simulink model "baseline"  (R2025b)
settings: Solver=ode45  StartTime=0.0  StopTime=0.1  MaxStep=1e-5  RelTol=1e-8  AbsTol=1e-10
model workspace (MAT data in the model file):
  F = 0.008
  J = 0.003
  L = 0.0085
  Rs = 0.2
  Udc = 250
  p = 4
  psi = 0.175
Description:
  | Lumped AFPM equivalent with ideal complementary gates [A+ A- B+ B- C+ C-]. w_ref is a test interface only.
settings Model: Creator=A  LastModifiedBy=A

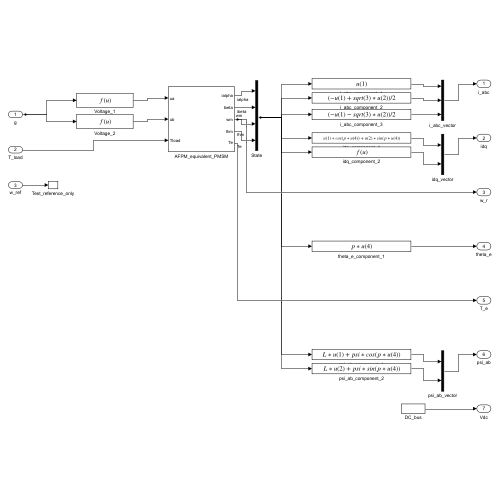
[thumbnail: Simulink's stored preview of the top-level diagram]
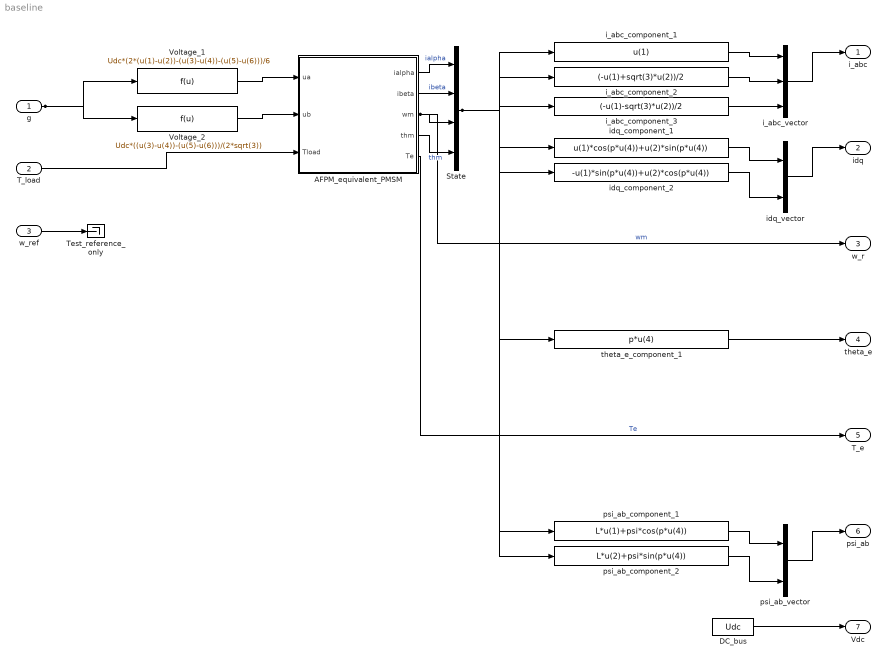
== system baseline ==
  g : Inport  Unit=1  PortDimensions=6
  T_load : Inport  Port=2  Unit=N*m  PortDimensions=1
  w_ref : Inport  Port=3  Unit=rpm  PortDimensions=1
  AFPM_equivalent_PMSM : Subsystem
  DC_bus : Constant  Value=Udc
  State : Mux
  Test_reference_only : Terminator
  Voltage_1 : Fcn  Expr=Udc*(2*(u(1)-u(2))-(u(3)-u(4))-(u(5)-u(6)))/6
  Voltage_2 : Fcn  Expr=Udc*((u(3)-u(4))-(u(5)-u(6)))/(2*sqrt(3))
  i_abc_component_1 : Fcn  Expr=u(1)
  i_abc_component_2 : Fcn  Expr=(-u(1)+sqrt(3)*u(2))/2
  i_abc_component_3 : Fcn  Expr=(-u(1)-sqrt(3)*u(2))/2
  i_abc_vector : Mux  Inputs=3
  idq_component_1 : Fcn  Expr=u(1)*cos(p*u(4))+u(2)*sin(p*u(4))
  idq_component_2 : Fcn  Expr=-u(1)*sin(p*u(4))+u(2)*cos(p*u(4))
  idq_vector : Mux  Inputs=2
  psi_ab_component_1 : Fcn  Expr=L*u(1)+psi*cos(p*u(4))
  psi_ab_component_2 : Fcn  Expr=L*u(2)+psi*sin(p*u(4))
  psi_ab_vector : Mux  Inputs=2
  theta_e_component_1 : Fcn  Expr=p*u(4)
  i_abc : Outport  Unit=A
  idq : Outport  Port=2  Unit=A
  w_r : Outport  Port=3  Unit=rad/s
  theta_e : Outport  Port=4  Unit=rad
  T_e : Outport  Port=5  Unit=N*m
  psi_ab : Outport  Port=6  Unit=Wb
  Vdc : Outport  Port=7  Unit=V
  wires:
  w_ref/1 -> Test_reference_only/1
  g/1 -> Voltage_1/1, Voltage_2/1
  Voltage_1/1 -> AFPM_equivalent_PMSM/1(ua)
  Voltage_2/1 -> AFPM_equivalent_PMSM/2(ub)
  T_load/1 -> AFPM_equivalent_PMSM/3(Tload)
  AFPM_equivalent_PMSM/1(ialpha) -> State/1  "ialpha"
  AFPM_equivalent_PMSM/2(ibeta) -> State/2  "ibeta"
  AFPM_equivalent_PMSM/3(wm) -> State/3, w_r/1  "wm"
  AFPM_equivalent_PMSM/4(thm) -> State/4  "thm"
  State/1 -> i_abc_component_1/1, i_abc_component_2/1, i_abc_component_3/1, idq_component_1/1, idq_component_2/1, theta_e_component_1/1, psi_ab_component_1/1, psi_ab_component_2/1
  i_abc_component_1/1 -> i_abc_vector/1
  i_abc_component_2/1 -> i_abc_vector/2
  i_abc_component_3/1 -> i_abc_vector/3
  i_abc_vector/1 -> i_abc/1
  idq_component_1/1 -> idq_vector/1
  idq_component_2/1 -> idq_vector/2
  idq_vector/1 -> idq/1
  theta_e_component_1/1 -> theta_e/1
  AFPM_equivalent_PMSM/5(Te) -> T_e/1  "Te"
  psi_ab_component_1/1 -> psi_ab_vector/1
  psi_ab_component_2/1 -> psi_ab_vector/2
  psi_ab_vector/1 -> psi_ab/1
  DC_bus/1 -> Vdc/1

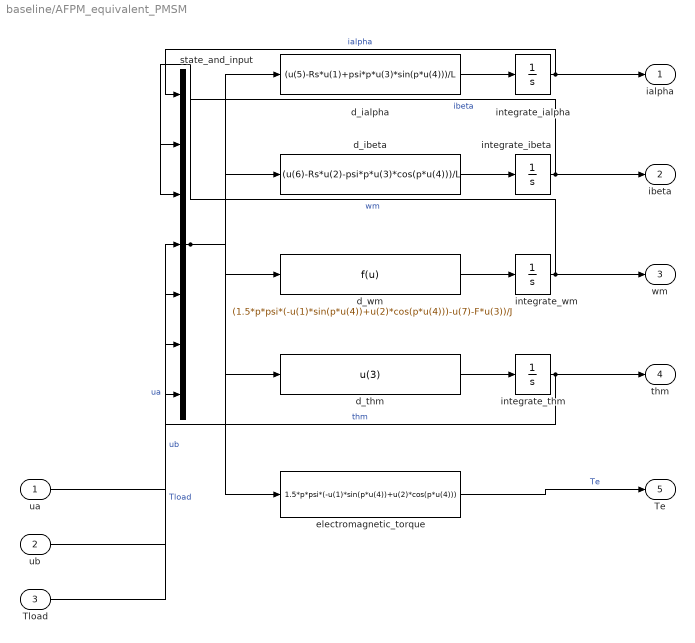
== system baseline/AFPM_equivalent_PMSM ==
  ua : Inport  Unit=V
  ub : Inport  Port=2  Unit=V
  Tload : Inport  Port=3  Unit=N*m
  d_ialpha : Fcn  Expr=(u(5)-Rs*u(1)+psi*p*u(3)*sin(p*u(4)))/L
  d_ibeta : Fcn  Expr=(u(6)-Rs*u(2)-psi*p*u(3)*cos(p*u(4)))/L
  d_thm : Fcn  Expr=u(3)
  d_wm : Fcn  Expr=(1.5*p*psi*(-u(1)*sin(p*u(4))+u(2)*cos(p*u(4)))-u(7)-F*u(3))/J
  electromagnetic_torque : Fcn  Expr=1.5*p*psi*(-u(1)*sin(p*u(4))+u(2)*cos(p*u(4)))
  integrate_ialpha : Integrator
  integrate_ibeta : Integrator
  integrate_thm : Integrator
  integrate_wm : Integrator
  state_and_input : Mux  Inputs=7
  ialpha : Outport  Unit=A
  ibeta : Outport  Port=2  Unit=A
  wm : Outport  Port=3  Unit=rad/s
  thm : Outport  Port=4  Unit=rad
  Te : Outport  Port=5  Unit=N*m
  wires:
  electromagnetic_torque/1 -> Te/1  "Te"
  Tload/1 -> state_and_input/7  "Tload"
  ub/1 -> state_and_input/6  "ub"
  ua/1 -> state_and_input/5  "ua"
  integrate_thm/1 -> state_and_input/4, thm/1  "thm"
  d_thm/1 -> integrate_thm/1
  integrate_wm/1 -> state_and_input/3, wm/1  "wm"
  d_wm/1 -> integrate_wm/1
  integrate_ibeta/1 -> state_and_input/2, ibeta/1  "ibeta"
  d_ibeta/1 -> integrate_ibeta/1
  integrate_ialpha/1 -> state_and_input/1, ialpha/1  "ialpha"
  d_ialpha/1 -> integrate_ialpha/1
  state_and_input/1 -> electromagnetic_torque/1, d_thm/1, d_wm/1, d_ibeta/1, d_ialpha/1
